simulink model "dc_motor_pid_diffeq"  (R2026a)
settings: Solver=ode45  StopTime=5  MaxStep=0.001  RelTol=1e-08  AbsTol=1e-10
model workspace (MAT data in the model file):
  A = [-4  -0.2; 3.33333333333  -0.0333333333333]
  B = [2  0; 0  -33.3333333333]
  C = [0  1; 1  0]
  D = [0  0; 0  0]
  Kb = 4.93696219862
  Kd = 1.84809830698
  Ki = 45.0448010417
  Kp = 17.9594547575
  Nf = 194.356054433
  Reference = 100
  TorqueTime = 1
  TorqueValue = 0
  VinValue = 12
  Vmax = 48
  Vmin = -48
  beta = 1
  gamma = 0
  p.Ra = 2
  p.La = 0.5
  p.Kt = 0.1
  p.Ke = 0.1
  p.Jm = 0.01
  p.Bm = 0.001
  p.JL = 0.02
  p.J = 0.03
  p.B = 0.001
  p.w_ref = 100
  p.Vmin = -48
  p.Vmax = 48
  p.beta = 1
  p.gamma = 0
  p.derivativeRatio = 20
  p.minimumFilterTime = 0.001
  p.ts_spec = 2
  p.os_spec = 5
  p.ess_spec = 0.2
  p.band = 0.02
  p.dt = 0.001
  p.RelTol = 1e-08
  p.AbsTol = 1e-10
  p.seed = 7
  p.Tsim = 5
  p.Tsim_ol = 30
  p.TL_step = 0.05
  p.TL_time = 1
  p.config.schemaVersion = 1
  p.config.physical.Ra = 2
  p.config.physical.La = 0.5
  p.config.physical.Kt = 0.1
  p.config.physical.Ke = 0.1
  p.config.physical.Jm = 0.01
  p.config.physical.Bm = 0.001
  p.config.physical.JL = 0.02
  p.config.control.reference = 100
  p.config.control.Vmin = -48
  p.config.control.Vmax = 48
  p.config.control.beta = 1
  p.config.control.gamma = 0
  p.config.control.derivativeRatio = 20
  p.config.control.minimumFilterTime = 0.001
  p.config.control.antiWindup = 'back-calculation'
  p.config.chosenTargets.settlingBand = 0.02
  p.config.chosenTargets.settlingTime = 2
  p.config.chosenTargets.overshootPercent = 5
  p.config.chosenTargets.steadyError = 0.2
  p.config.numerics.relativeTolerance = 1e-08
  p.config.numerics.absoluteTolerance = 1e-10
  p.config.numerics.outputStep = 0.001
  p.config.numerics.seed = 7
  p.config.assumptions = {'Bipolar +/-48 V is an engineering choice; the assignment specifies no voltage limit.'; 'Overshoot <=5% and steady error <=0.2 rad/s are chosen targets, not instructor-specified limits.'; 'The rigid load adds inertia only. Positive load torque opposes positive rotation.'}
  x0 = [0; 0]
libraries: slpidlib x1
settings Model: Creator=ievge  LastModifiedBy=ievge

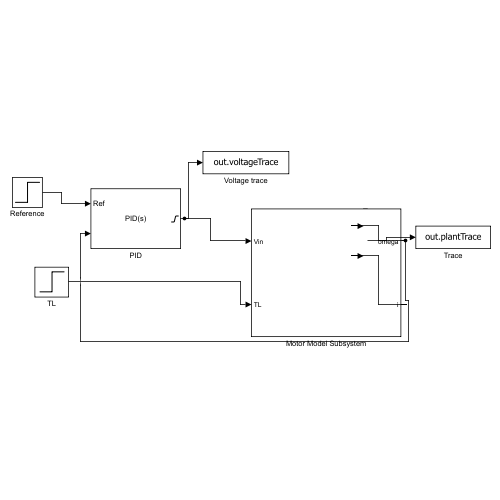
[thumbnail: Simulink's stored preview of the top-level diagram]
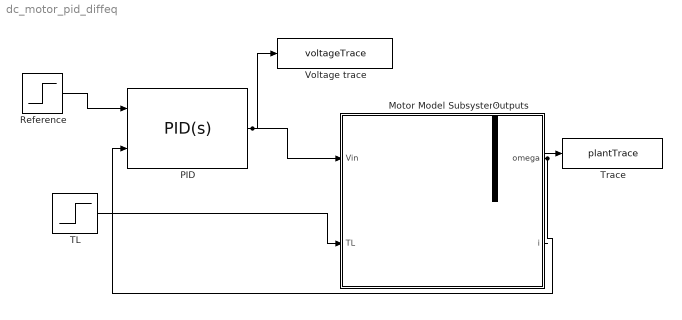
== system dc_motor_pid_diffeq ==
  Motor Model Subsystem : Subsystem
  Outputs : Mux  Inputs=2
  PID : slpidlib/PID Controller (2DOF)  Controller=PID  Form=Parallel  TimeDomain=Continuous-time  UseExternalTs=off  SampleTime=-1  IntegratorMethod=Forward Euler  FilterMethod=Forward Euler  ControllerParametersSource=internal  P=Kp  I=Ki  UseKiTs=off  D=Kd  UseExternalDerivativeSource=off  N=Nf  UseFilter=on  b=beta  c=gamma  TunerSelectOption=Transfer Function Based (PID Tuner App)  InitialConditionSource=internal  InitialConditionForIntegrator=0  InitialConditionForFilter=0  DifferentiatorICPrevScaledInput=0  ExternalReset=none  TrackingMode=off  Kt=1  LimitOutput=on  SatLimitsSource=internal  UpperSaturationLimit=Vmax  LowerSaturationLimit=Vmin  LinearizeAsGain=on  AntiWindupMode=back-calculation  Kb=Kb  LimitIntegrator=off  UpperIntegratorSaturationLimit=inf  LowerIntegratorSaturationLimit=-inf  POutMin=[]  POutMax=[]  IOutMin=[]  IOutMax=[]  DOutMin=[]  DOutMax=[]  NOutMin=[]  NOutMax=[]  bOutMin=[]  bOutMax=[]  cOutMin=[]  cOutMax=[]  SumOutMin=[]  SumOutMax=[]  SaturationOutMin=[]  SaturationOutMax=[]  PParamMin=[]  PParamMax=[]  IParamMin=[]  IParamMax=[]  DParamMin=[]  DParamMax=[]  NParamMin=[]  NParamMax=[]  bParamMin=[]  bParamMax=[]  cParamMin=[]  cParamMax=[]  KbParamMin=[]  KbParamMax=[]  KtParamMin=[]  KtParamMax=[]  KbOutMin=[]  KbOutMax=[]  KtOutMin=[]  KtOutMax=[]  IntegratorOutMin=[]  IntegratorOutMax=[]  FilterOutMin=[]  FilterOutMax=[]  SumI1OutMin=[]  SumI1OutMax=[]  SumI2OutMin=[]  SumI2OutMax=[]  SumI3OutMin=[]  SumI3OutMax=[]  SumI4OutMin=[]  SumI4OutMax=[]  SumDOutMin=[]  SumDOutMax=[]  Sum1OutMin=[]  Sum1OutMax=[]  Sum2OutMin=[]  Sum2OutMax=[]  Sum3OutMin=[]  Sum3OutMax=[]  DifferentiatorOutMin=[]  DifferentiatorOutMax=[]  FilterDiffOutCoefMin=[]  FilterDiffOutCoefMax=[]  ReciprocalOutMin=[]  ReciprocalOutMax=[]  SumDenOutMin=[]  SumDenOutMax=[]  SumNumOutMin=[]  SumNumOutMax=[]  DivideOutMin=[]  DivideOutMax=[]  UdiffTsProdOutMin=[]  UdiffTsProdOutMax=[]  NTsProdOutMin=[]  NTsProdOutMax=[]  UintegralTsProdOutMin=[]  UintegralTsProdOutMax=[]  UngainTsProdOutMin=[]  UngainTsProdOutMax=[]  ClampingZeroOutDataTypeStr=Inherit: Inherit via back propagation  ClampingZeroOutMin=[]  ClampingZeroOutMax=[]  FilterDenConstantOutDataTypeStr=Inherit: Inherit via back propagation  FilterDenConstantOutMin=[]  FilterDenConstantOutMax=[]  PCopyOutDataTypeStr=Inherit: Inherit via back propagation  PCopyOutMin=[]  PCopyOutMax=[]  NCopyOutDataTypeStr=Inherit: Inherit via back propagation  NCopyOutMin=[]  NCopyOutMax=[]  IntegratorContinuousStateAttributes=''  IntegratorStateMustResolveToSignalObject=off  IntegratorRTWStateStorageClass=Auto  FilterContinuousStateAttributes=''  FilterStateMustResolveToSignalObject=off  FilterRTWStateStorageClass=Auto  ParallelPVariant=InternalParameters  IdealPVariant=Disabled  IVariant=InternalParameters  DVariant=InternalParameters  bVariant=InternalParameters  cVariant=InternalParameters  IntegratorVariant=Continuous  SatVariant=Enabled  AWVariant=BackCalculation  PCopyVariant=Disabled  TRVariant=Disabled  FdbkBlocksVariant=Forward  IdealPFdbkVariant=Disabled  SatFdbkVariant=Disabled  DerivativeFilterVariant=ContFilter  NVariant=InternalParameters  NCopyVariant=Disabled  FilterICVariant=InternalICsFilter  IntegratorICVariant=InternalICs  ExternalResetVariant=Disabled  TRSumVariant=Passthrough  SumFdbkVariant=Disabled  SumVariant=Sum_PID  TsampFilterVariant=InternalTs  TsampNgainVariant=Passthrough  TsampIntegralVariant=Disabled_SignalSpec  ExternalSaturationOutDataTypeStr=Inherit: Same as second input  DerivativeSourceVariant=ErrorSignal  PreIntVariant=InternalPreInt
  Reference : Step  Time=0  FinalValue=Reference  SampleTime=0
  TL : Step  Time=TorqueTime  FinalValue=TorqueValue  SampleTime=0
  Trace : ToWorkspace  VariableName=plantTrace  SaveFormat=Timeseries  SampleTime=-1
  Voltage trace : ToWorkspace  VariableName=voltageTrace  SaveFormat=Timeseries  SampleTime=-1
  wires:
  Outputs/1 -> Trace/1
  Reference/1 -> PID/1
  Motor Model Subsystem/1(omega) -> PID/2, Outputs/1
  PID/1 -> Motor Model Subsystem/1(Vin), Voltage trace/1
  TL/1 -> Motor Model Subsystem/2(TL)
  Motor Model Subsystem/2(i) -> Outputs/2

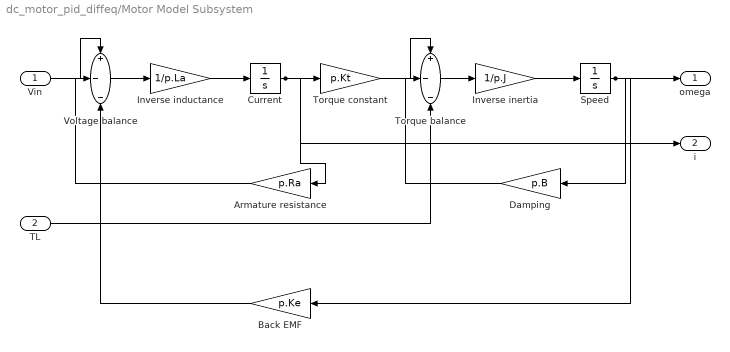
== system dc_motor_pid_diffeq/Motor Model Subsystem ==
  Vin : Inport
  TL : Inport  Port=2
  Armature resistance : Gain  Gain=p.Ra
  Back EMF : Gain  Gain=p.Ke
  Current : Integrator  InitialCondition=x0(1)
  Damping : Gain  Gain=p.B
  Inverse inductance : Gain  Gain=1/p.La
  Inverse inertia : Gain  Gain=1/p.J
  Speed : Integrator  InitialCondition=x0(2)
  Torque balance : Sum  Inputs=+--
  Torque constant : Gain  Gain=p.Kt
  Voltage balance : Sum  Inputs=+--
  omega : Outport
  i : Outport  Port=2
  wires:
  TL/1 -> Torque balance/3
  Damping/1 -> Torque balance/2
  Back EMF/1 -> Voltage balance/3
  Armature resistance/1 -> Voltage balance/2
  Speed/1 -> Damping/1, Back EMF/1, omega/1
  Inverse inertia/1 -> Speed/1
  Torque balance/1 -> Inverse inertia/1
  Torque constant/1 -> Torque balance/1
  Current/1 -> Armature resistance/1, i/1, Torque constant/1
  Inverse inductance/1 -> Current/1
  Voltage balance/1 -> Inverse inductance/1
  Vin/1 -> Voltage balance/1
